simulink model "GCS_MVP_AI"  (R2026b)
settings: Solver=ode4  StopTime=90  FixedStep=0.005
values from neighbouring files (symbols this model uses):
  MVP = 0.02    [QuadInterfaces_AI.sldd]
settings Model: DataDictionary=QuadInterfaces_AI.sldd  Creator=JonathanTee  LastModifiedBy=JonathanTee
settings ModelReferenceCC: ModelReferenceMinAlgLoopOccurrences=on

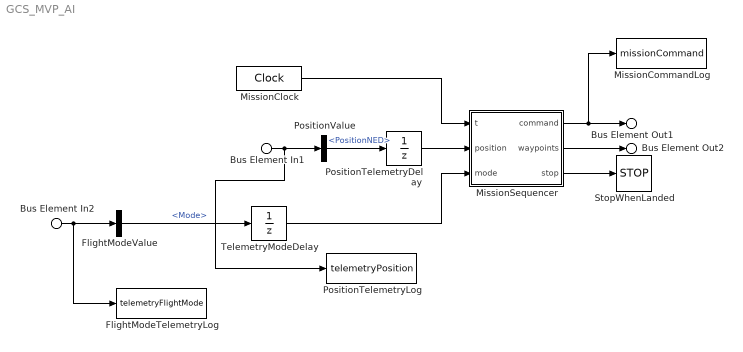
== system GCS_MVP_AI ==
  Bus Element In1 : Inport  PortName=Position
  Bus Element In2 : Inport  Port=2  PortName=FlightMode
  FlightModeTelemetryLog : ToWorkspace  VariableName=telemetryFlightMode  SaveFormat=Timeseries  SampleTime=-1
  FlightModeValue : BusSelector  OutputSignals=Mode
  MissionClock : DigitalClock  SampleTime=MVP.SampleTime
  MissionCommandLog : ToWorkspace  VariableName=missionCommand  SaveFormat=Timeseries  SampleTime=-1
  MissionSequencer : MATLAB Function  TreatAsAtomicUnit=on
  PositionTelemetryDelay : UnitDelay  InitialCondition=MVP.InitialPosition  SampleTime=MVP.SampleTime
  PositionTelemetryLog : ToWorkspace  VariableName=telemetryPosition  SaveFormat=Timeseries  SampleTime=-1
  PositionValue : BusSelector  OutputSignals=PositionNED
  StopWhenLanded : Stop
  TelemetryModeDelay : UnitDelay  SampleTime=MVP.SampleTime
  Bus Element Out1 : Outport  PortName=MissionCommand
  Bus Element Out2 : Outport  Port=2  PortName=WaypointTargets
  wires:
  FlightModeValue/1 -> TelemetryModeDelay/1  "<Mode>"
  Bus Element In2/1 -> FlightModeTelemetryLog/1, FlightModeValue/1
  PositionTelemetryDelay/1 -> MissionSequencer/2(position)
  PositionValue/1 -> PositionTelemetryDelay/1  "<PositionNED>"
  MissionSequencer/1(command) -> MissionCommandLog/1, Bus Element Out1/1
  Bus Element In1/1 -> PositionValue/1, PositionTelemetryLog/1
  MissionClock/1 -> MissionSequencer/1(t)
  TelemetryModeDelay/1 -> MissionSequencer/3(mode)
  MissionSequencer/2(waypoints) -> Bus Element Out2/1
  MissionSequencer/3(stop) -> StopWhenLanded/1

== matlab function GCS_MVP_AI/MissionSequencer ==
  settings: updateMethod=DISCRETE  sampleTime=MVP.SampleTime
  data: t input; command output Bus: MissionCommand_IF; position input double size=[3 1]; mode input; waypoints output Bus: WaypointTargets_IF; stop output
function [command,waypoints,stop]=gcs(t,position,mode)
%#codegen
fm.Mode=mode;
pos.PositionNED=position;
[command,waypoints,stop]=stage02_gcs(t,pos,fm);
end
